simulink model "A3"  (R2025b)
settings: Solver=FixedStepAuto  StartTime=0.0  StopTime=2  RelTol=1e-3
libraries: androidaudiovideolib x1, dspfdesign x1, dspstat3 x1, dspadpt3 x1, androidcommunicationlib x1
settings Model: Creator=vishr  LastModifiedBy=vishr
settings OptimizationCC: DefaultParameterBehavior=Inlined  EnhancedBackFolding=on  PassReuseOutputArgsAs=Individual arguments  ZeroExternalMemoryAtStartup=off  ZeroInternalMemoryAtStartup=off  MaxStackSize=64  OptimizeBlockOrder=speed  DifferentSizesBufferReuse=on  OptimizationCustomize=off  EfficientTunableParamExpr=on
settings DebuggingCC: ParameterTunabilityLossMsg=error
settings HardwareCC: ProdBitPerPointer=32.0  ProdBitPerSizeT=32.0  ProdBitPerPtrDiffT=32.0  ProdLargestAtomicInteger=Long  ProdLargestAtomicFloat=Double  ProdWordSize=32.0  ProdHWDeviceType=ARM Compatible->ARM Cortex-A (32-bit)
settings SFSimCC: MATLABDynamicMemAlloc=off
settings RTWCC: SystemTargetFile=ert.tlc  HardwareBoard=Android Device  TLCOptions="-aInlineSetEventsForThisBaseRateFcn=TLC_FALSE -aSuppressMultiTaskScheduler=TLC_FALSE  -aRateBasedStepFcn=0"  TemplateMakefile=ert_default_tmf  RTWVerbose=off  Toolchain=Android SDK/NDK Tools  Description=Embedded Coder
settings CodeAppCC: ForceParamTrailComments=on  IgnoreCustomStorageClasses=off  OperatorAnnotations=on  SimulinkDataObjDesc=on  SFDataObjDesc=on  InsertBlockDesc=on

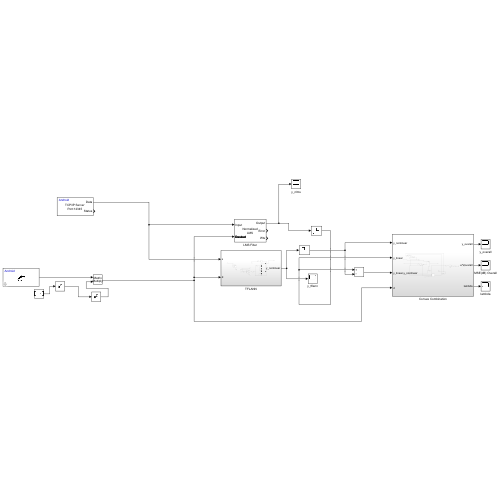
[thumbnail: Simulink's stored preview of the top-level diagram]
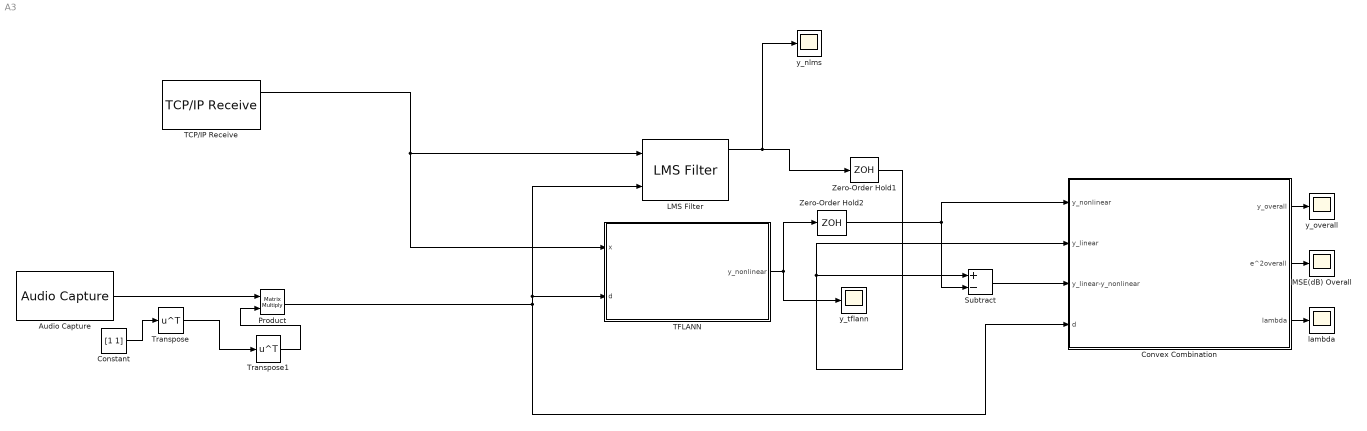
== system A3 ==
  Audio Capture : androidaudiovideolib/Audio Capture  SampleFreq=44100  FrameSize=4410  SampleTime=0.1  SimulateUsing=Code generation  DeviceStr=0  QueueDuration=0  BlockPlatform=Android  AudioSamplingFreq=44100
  Constant : Constant  Value=[1 1]
  Convex Combination : Subsystem
  LMS Filter : dspadpt3/LMS Filter  Algo=Normalized LMS  L=10  stepflag=Dialog  mu=0.1  leakage=1.0  ic=0  Adapt=off  resetflag=None  weights=on  addnparflag=off  roundingMode=Floor  overflowMode=off  secondCoeffMode=Binary point scaling  secondCoeffWordLength=2  secondCoeffFracLength=15  prodOutput2Mode=Binary point scaling  prodOutput2FracLength=20  prodOutput3Mode=Binary point scaling  prodOutput3FracLength=20  prodOutput4Mode=Binary point scaling  prodOutput4FracLength=20  quotientMode=Binary point scaling  quotientFracLength=20  accum2Mode=Binary point scaling  accum2FracLength=20
      settings: LibrarySourceBlock=dsphdlsupportfiltering/LMS Filter
  MSE(dB) Overall : Scope
      settings: ActiveDisplayYMinimum=-19.468077474449345  ActiveDisplayYMaximum=2.1621493055710039  DataLoggingVariableName=ScopeData8
  Product : Product  Multiplication=Matrix(*)
  Subtract : Sum  Inputs=+-
  TCP/IP Receive : androidcommunicationlib/TCP//IP Receive  TCPReceiveId=A3/TCP//IP_Receive  Mode_=Server  LocalServerPort_=12345  RemoteAddr_=127.0.0.1  RemoteServerPort_=25000  DataType_=double  DataSize_=4410  SampleTime_=1e-4  ClientPortBindingSelection_=off  ClientPortToBind_=35000  BlockingMode_=off  BlockTimeout_=0.1
  TFLANN : Subsystem
  Transpose : Math  Operator=transpose
  Transpose1 : Math  Operator=transpose
  Zero-Order Hold1 : ZeroOrderHold  SampleTime=1e-4
  Zero-Order Hold2 : ZeroOrderHold  SampleTime=1e-4
  lambda : Scope
      settings: ActiveDisplayYMinimum=-0.12499999999999997  ActiveDisplayYMaximum=1.125  DataLoggingVariableName=ScopeData9
  y_nlms : Scope
  y_overall : Scope
      settings: ActiveDisplayYMinimum=-3.93121235585972  ActiveDisplayYMaximum=4.0932209788377252  DataLoggingVariableName=ScopeData5
  y_tflann : Scope
      settings: ActiveDisplayYMinimum=-2.0302293992486709  ActiveDisplayYMaximum=2.2383486881688421
  wires:
  LMS Filter/1 -> y_nlms/1, Zero-Order Hold1/1
  TFLANN/1(y_nonlinear) -> y_tflann/1, Zero-Order Hold2/1
  Product/1 -> Convex Combination/4(d), LMS Filter/2, TFLANN/2(d)
  Constant/1 -> Transpose/1
  Transpose/1 -> Transpose1/1
  Audio Capture/1 -> Product/1
  Transpose1/1 -> Product/2
  TCP/IP Receive/1 -> TFLANN/1(x), LMS Filter/1
  Subtract/1 -> Convex Combination/3(y_linear-y_nonlinear)
  Zero-Order Hold1/1 -> Subtract/1, Convex Combination/2(y_linear)
  Zero-Order Hold2/1 -> Subtract/2, Convex Combination/1(y_nonlinear)
  Convex Combination/1(y_overall) -> y_overall/1
  Convex Combination/2(e^2overall) -> MSE(dB) Overall/1
  Convex Combination/3(lambda) -> lambda/1

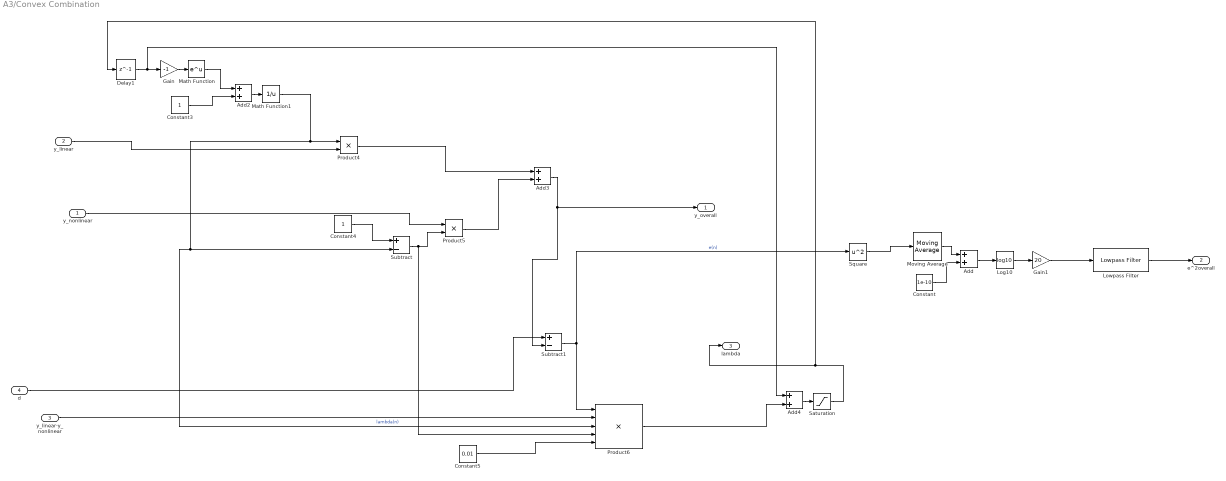
== system A3/Convex Combination ==
  y_nonlinear : Inport
  y_linear : Inport  Port=2
  y_linear-y_nonlinear : Inport  Port=3
  d : Inport  Port=4
  Add{,2..4} (4 alike) : Sum
  Constant : Constant  Value=1e-10
  Constant3 : Constant
  Constant4 : Constant
  Constant5 : Constant  Value=0.01
  Delay1 : Delay  DelayLength=1  InputProcessing=Columns as channels (frame based)
  Gain : Gain  Gain=-1
  Gain1 : Gain  Gain=20
  Log10 : Math  Operator=log10
  Lowpass Filter : dspfdesign/Lowpass Filter  FilterType=FIR  DesignForMinimumOrder=on  FilterOrder=50  PassbandFrequency=0.001  StopbandFrequency=0.03  PassbandRipple=0.1  StopbandAttenuation=80  SampleRateMode=Use normalized frequency (0 to 1)  SampleRate=44100  SimulateUsing=Interpreted execution  roundingMode=Floor  coeffsDataTypeStr=fixdt(1,16)
  Math Function : Math
  Math Function1 : Math  Operator=reciprocal
  Moving Average : dspstat3/Moving Average  Method=Sliding window  ForgettingFactorPort=off  SpecifyWindowLength=on  WindowLength=4  OverlapLength=3  AllowArbitraryInputLength=off  ForgettingFactor=0.9  SimulateUsing=Interpreted execution
  Product4 : Product
  Product5 : Product
  Product6 : Product  Inputs=5
  Saturation : Saturate  UpperLimit=0.732  LowerLimit=0
  Square : Math  Operator=square
  Subtract : Sum  Inputs=+-
  Subtract1 : Sum  Inputs=+-
  y_overall : Outport
  e^2overall : Outport  Port=2
  lambda : Outport  Port=3
  wires:
  Add2/1 -> Math Function1/1
  Math Function/1 -> Add2/1
  y_nonlinear/1 -> Product5/1
  Subtract1/1 -> Square/1, Product6/1  "e(n)"
  Product6/1 -> Add4/2
  Math Function1/1 -> Product4/1, Product6/3, Subtract/2  "lambda(n)"
  Subtract/1 -> Product6/4, Product5/2
  y_linear/1 -> Product4/2
  Saturation/1 -> lambda/1, Delay1/1
  Constant3/1 -> Add2/2
  Constant5/1 -> Product6/5
  Add3/1 -> y_overall/1, Subtract1/2
  Gain/1 -> Math Function/1
  Constant4/1 -> Subtract/1
  Product5/1 -> Add3/2
  Delay1/1 -> Add4/1, Gain/1
  Product4/1 -> Add3/1
  d/1 -> Subtract1/1
  y_linear-y_nonlinear/1 -> Product6/2
  Add4/1 -> Saturation/1
  Square/1 -> Moving Average/1
  Moving Average/1 -> Add/1
  Constant/1 -> Add/2
  Add/1 -> Log10/1
  Log10/1 -> Gain1/1
  Gain1/1 -> Lowpass Filter/1
  Lowpass Filter/1 -> e^2overall/1

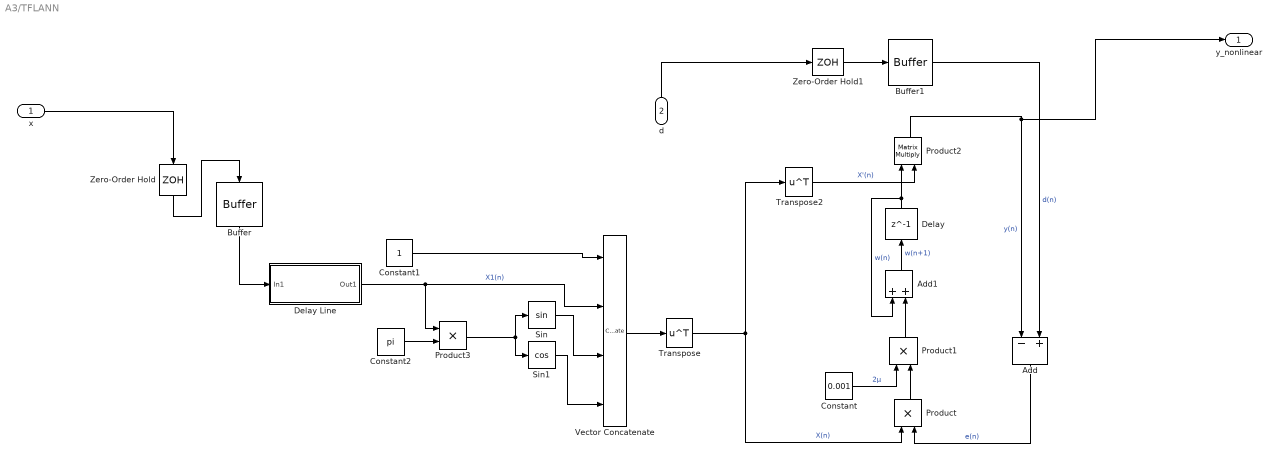
== system A3/TFLANN ==
  x : Inport
  d : Inport  Port=2
  Add : Sum  Inputs=-+
  Add1 : Sum
  Buffer : Buffer  N=1  OutputFrames=off
  Buffer1 : Buffer  N=1  OutputFrames=off
  Constant : Constant  Value=0.001
  Constant1 : Constant
  Constant2 : Constant  Value=pi
  Delay : Delay  DelayLength=1  InputProcessing=Columns as channels (frame based)
  Delay Line : Subsystem
  Product : Product
  Product1 : Product
  Product2 : Product  Multiplication=Matrix(*)
  Product3 : Product
  Sin : Trigonometry
  Sin1 : Trigonometry  Operator=cos
  Transpose : Math  Operator=transpose
  Transpose2 : Math  Operator=transpose
  Vector Concatenate : Concatenate  NumInputs=4
  Zero-Order Hold : ZeroOrderHold  SampleTime=1/(6e3)
  Zero-Order Hold1 : ZeroOrderHold  SampleTime=1/(6e3)
  y_nonlinear : Outport
  wires:
  Transpose2/1 -> Product2/2  "X'(n)"
  Add/1 -> Product/2  "e(n)"
  Delay Line/1(Out1) -> Vector Concatenate/2, Product3/1  "X1(n)"
  Sin1/1 -> Vector Concatenate/4
  Product1/1 -> Add1/2
  Product/1 -> Product1/2
  Delay/1 -> Add1/1, Product2/1  "w(n)"
  Sin/1 -> Vector Concatenate/3
  Vector Concatenate/1 -> Transpose/1
  Constant/1 -> Product1/1  "2μ"
  Add1/1 -> Delay/1  "w(n+1)"
  Product2/1 -> Add/1, y_nonlinear/1  "y(n)"
  Transpose/1 -> Transpose2/1, Product/1  "X(n)"
  Zero-Order Hold/1 -> Buffer/1
  Constant2/1 -> Product3/2
  Buffer1/1 -> Add/2  "d(n)"
  Product3/1 -> Sin/1, Sin1/1
  Constant1/1 -> Vector Concatenate/1
  Buffer/1 -> Delay Line/1(In1)
  Zero-Order Hold1/1 -> Buffer1/1
  x/1 -> Zero-Order Hold/1
  d/1 -> Zero-Order Hold1/1

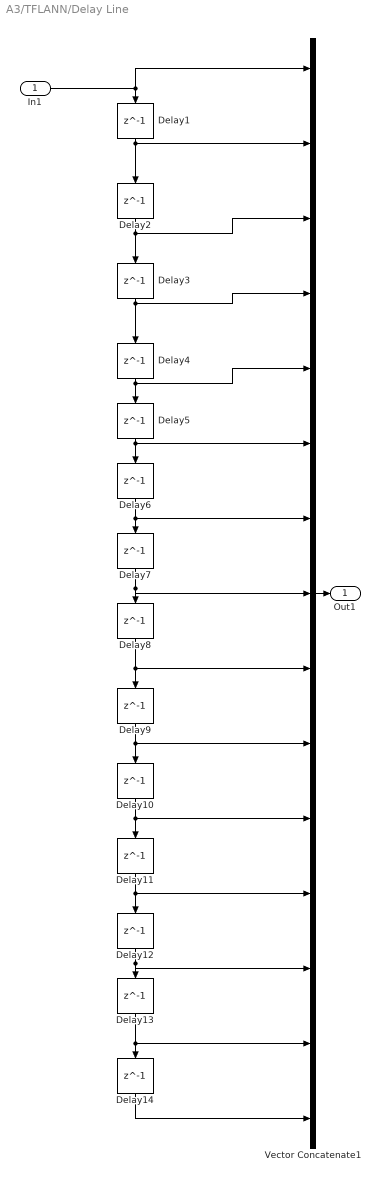
== system A3/TFLANN/Delay Line ==
  In1 : Inport
  Delay{1..14} (14 alike) : Delay  DelayLength=1  InputProcessing=Columns as channels (frame based)
  Vector Concatenate1 : Concatenate  NumInputs=15
  Out1 : Outport
  wires:
  Delay14/1 -> Vector Concatenate1/15
  Delay5/1 -> Delay6/1, Vector Concatenate1/6
  Delay6/1 -> Delay7/1, Vector Concatenate1/7
  Delay3/1 -> Delay4/1, Vector Concatenate1/4
  Delay8/1 -> Delay9/1, Vector Concatenate1/9
  Delay12/1 -> Vector Concatenate1/13, Delay13/1
  In1/1 -> Delay1/1, Vector Concatenate1/1
  Delay13/1 -> Vector Concatenate1/14, Delay14/1
  Delay7/1 -> Delay8/1, Vector Concatenate1/8
  Delay11/1 -> Vector Concatenate1/12, Delay12/1
  Delay2/1 -> Delay3/1, Vector Concatenate1/3
  Delay9/1 -> Delay10/1, Vector Concatenate1/10
  Delay4/1 -> Vector Concatenate1/5, Delay5/1
  Delay1/1 -> Delay2/1, Vector Concatenate1/2
  Delay10/1 -> Delay11/1, Vector Concatenate1/11
  Vector Concatenate1/1 -> Out1/1
